simulink subsystem "sandBattery"  (R2023b)
settings: Solver=VariableStepAuto  StartTime=0.0  StopTime=10.0  RelTol=1e-3
values from neighbouring files (symbols this model uses):
  TES = struct()    [SetupTestHarness.m]    (also in ThermalBatterySetParam.m)
libraries: fl_lib x3, ee_lib x1, nesl_utility x1
settings Model: Creator=shachind  LastModifiedBy=shachind
settings OptimizationCC: ReuseModelBlockBuffer=off

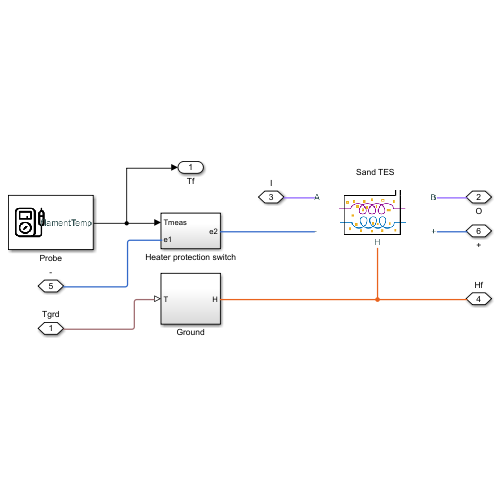
[thumbnail: Simulink's stored preview of the top-level diagram]
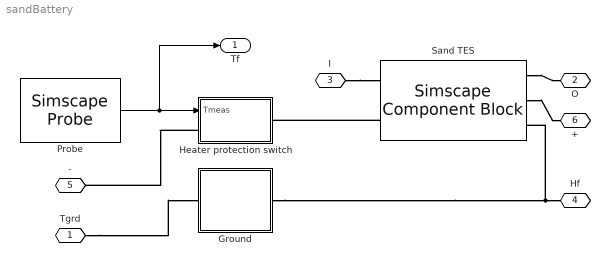
== system sandBattery ==
  Ground : Subsystem
  Heater protection switch : Subsystem
  Probe : SimscapeProbe  BoundBlock=10  Variables={filamentTemp}
  Sand TES : SimscapeComponentBlock  SourceFile=lumpedTES  ComponentPath=lumpedTES  ComponentVariants="[\"lumpedTES\"]"  ComponentVariantNames="[\"lumpedTES\"]"  ClassName=lumpedTES  SchemaVersion=1  coilShape=layoutShape.HelicalCoil  numCoilX=TES.numCoilX  numCoilY=TES.numCoilY  cellRefT=TES.cellRefT K  coilWidthHeater=TES.coilWidthHeater m  coilDiameterHeater=0.1 m  coilDepthHeater=TES.coilDepthHeater m  nturnsHeater=TES.nTrnsHeater  heaterTubeDia=TES.heaterTubeDia m  heaterTimeconst=TES.heaterTimeconst s  heaterRes=TES.heaterRes Ohm  heaterEmissivity=TES.heaterEmissivity  heaterMaxT=TES.heaterMaxT degC  coilWidthCooler=TES.coilWidthCooler m  coilDiameterCooler=0.1 m  coilDepthCooler=TES.coilDepthCooler m  nturnsCooler=TES.nTrnsCooler  pipeHydraulicDia=TES.pipeHydraulicDia m  sandDensity=TES.sandDensity kg/m^3  sandThCond=TES.sandThCond W/(K*m)  sandSpHeat=TES.sandSpHeat J/(K*kg)  sandInitT=TES.initTemp_degC degC  stfBtz=5.670374419e-8 W/(K^4*m^2)  biotFactor=7.04  filamentTemp_specify=off  filamentTemp_priority=None  filamentTemp=298.15 K  filamentTemp_nominal_specify=off  filamentTemp_nominal_unit=K  filamentTemp_nominal_value=1
      settings: CopyFcn=simscape.engine.sli.internal.componentblockcallback(gcbh,'COPY')  PreCopyFcn=simscape.engine.sli.internal.componentblockcallback(gcbh,'PRECOPY')  PreDeleteFcn=simscape.engine.sli.internal.componentblockcallback(gcbh,'PREDELETE')  InternalSimscapePortConfiguration="{\"Bottom\":[{\"id\":\"H\",\"label\":\"H\",\"type\":\"foundation.thermal.thermal\"}],\"Left\":[{\"id\":\"A\",\"label\":\"A\",\"type\":\"foundation.moist_air.moist_air\"},{\"id\":\"n\",\"label\":\"-\",\"type\":\"foundation.electrical.electrical\"}],\"Right\":[{\"id\":\"B\",\"label\":\"B\",\"type\":\"foundation.moist_air.moist_air\"},{\"id\":\"p\",\"label\":\"+\",\"type\":\"foundation.electrical.electrical\"}],\"Top\":[]}"
      mask Type: TES
  Tgrd : PMIOPort  Side=Left
  O : PMIOPort  Port=2  Side=Left
  I : PMIOPort  Port=3  Side=Left
  Hf : PMIOPort  Port=4  Side=Left
  - : PMIOPort  Port=5  Side=Left
  + : PMIOPort  Port=6  Side=Left
  Tf : Outport
  wires:
  Probe/1 -> Heater protection switch/1(Tmeas), Tf/1
  connections:
  Hf/RConn1 -- Sand TES/RConn3 -- Ground/LConn1
  Sand TES/RConn1 -- O/RConn1
  Sand TES/RConn2 -- +/RConn1
  I/RConn1 -- Sand TES/LConn1
  Tgrd/RConn1 -- Ground/RConn1
  Sand TES/LConn2 -- Heater protection switch/RConn1
  Heater protection switch/LConn1 -- -/RConn1

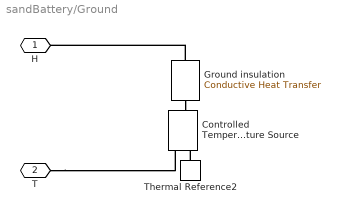
== system sandBattery/Ground ==
  Controlled Temperature Source : fl_lib/Thermal/Thermal Sources/Controlled Temperature Source
  Ground insulation : fl_lib/Thermal/Thermal Elements/Conductive Heat Transfer  thermal_type=foundation.enum.ConstantVariableTabulated.Constant  wall_geometry=foundation.enum.ConductionWallGeometry.Planar  area=200.2374 m^2  thickness=0.2 m  d_in=0.05 m  d_out=0.1 m  L=1 m  th_cond_min=10 W/(K*m)  th_cond=0.025 W/(K*m)  th_cond_TLU=[413, 401, 392, 383, 371, 357, 342] W/(K*m)  temp_TLU=[200, 273, 400, 600, 800, 1000, 1200] K  T_specify=off  T_priority=None  T=0 K  T_nominal_specify=off  T_nominal_unit=K  T_nominal_value=1  Q_specify=off  Q_priority=None  Q=0 W  Q_nominal_specify=off  Q_nominal_unit=W  Q_nominal_value=1
  Thermal Reference2 : fl_lib/Thermal/Thermal Elements/Thermal Reference
  H : PMIOPort  Side=Left
  T : PMIOPort  Port=2  Side=Right
  connections:
  Ground insulation/LConn1 -- H/RConn1
  Ground insulation/RConn1 -- Controlled Temperature Source/LConn1
  Thermal Reference2/LConn1 -- Controlled Temperature Source/RConn2
  T/RConn1 -- Controlled Temperature Source/RConn1

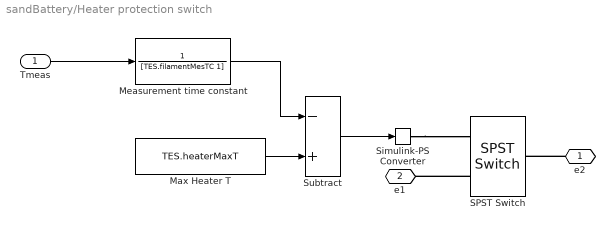
== system sandBattery/Heater protection switch ==
  Tmeas : Inport
  Max Heater T : Constant  Value=TES.heaterMaxT
  Measurement time constant : TransferFcn  Denominator=[TES.filamentMesTC 1]
  SPST Switch : ee_lib/Switches & Breakers/SPST Switch  R_closed=0.001 Ohm  G_open=1e-6 S  Threshold=10 V  Width=5 V  model_dynamics=1  t_on=10 s  t_off=10 s  initial_vT=0 V
      settings: InternalSimscapePortConfiguration="{\"Bottom\":[],\"Left\":[{\"id\":\"vT\",\"label\":\"vT\",\"type\":\"input\"},{\"id\":\"p\",\"label\":\"\",\"type\":\"foundation.electrical.electrical\"}],\"Right\":[{\"id\":\"n\",\"label\":\"\",\"type\":\"foundation.electrical.electrical\"}],\"Top\":[]}"
  Simulink-PS Converter : nesl_utility/Simulink-PS Converter  PhysicalDomain=network_engine_domain  SubClassName=ps_input  LeftPortType=input  RightPortType=output  PseudoPeriodic=off  Frequencies=[]  NoiseDistribution=none  NoiseParameters=[]  Unit=1  AffineConversion=off  FilteringAndDerivatives=provide  SimscapeFilterOrder=1  InputFilterTimeConstant=0.001  UdotUserProvided=0
  Subtract : Sum  Inputs=-+
  e2 : PMIOPort  Side=Right
  e1 : PMIOPort  Port=2  Side=Left
  wires:
  Subtract/1 -> Simulink-PS Converter/1
  Max Heater T/1 -> Subtract/2
  Measurement time constant/1 -> Subtract/1
  Tmeas/1 -> Measurement time constant/1
  connections:
  Simulink-PS Converter/RConn1 -- SPST Switch/LConn1
  SPST Switch/LConn2 -- e1/RConn1
  e2/RConn1 -- SPST Switch/RConn1
